simulink model "ps_25V_12kA_r"  (R2026b)
settings: Solver=ode23tb  StopTime=param.sim.simlength  FixedStep=param.glb_time.tc  MaxStep=param.glb_time.tc
values from neighbouring files (symbols this model uses):
  param = struct()    [init_model.m]
undefined symbols (not defined in the file or in its folder): magnitude
libraries: fl_lib x106, nesl_utility x71, afe_uvw_ctrl x5, ee_legacy_lib x5, discrete_time_low_pass_filter x2, three_windings_transformer x2, pi_ctrl x2, threephase_inductor_lib x1, dclink_for_two_levels x1, three_phase_pwm_modulator x1, three_phase_inverter_ideal_switch_based_model x1, three_phase_inverter_igbt_advanced_thermal_model x1
(part 2 of 5)

== system ps_25V_12kA_r/grid/grid_emulator ==
  3ph_Dyg_ssc : Subsystem
  Bus Selector : BusSelector  OutputSignals=ua_grid_emu,ub_grid_emu,uc_grid_emu
  Bus Selector1 : BusSelector  OutputSignals=gamma_grid_emulator,omega_grid_emulator
  Controlled Voltage Source : fl_lib/Electrical/Electrical Sources/Controlled Voltage Source
  Controlled Voltage Source1 : fl_lib/Electrical/Electrical Sources/Controlled Voltage Source
  Controlled Voltage Source2 : fl_lib/Electrical/Electrical Sources/Controlled Voltage Source
  Electrical Reference : fl_lib/Electrical/Electrical Elements/Electrical Reference
  Simulink-PS Converter : nesl_utility/Simulink-PS Converter  PhysicalDomain=network_engine_domain  SubClassName=ps_input  LeftPortType=input  RightPortType=output  PseudoPeriodic=off  Frequencies=[]  NoiseDistribution=none  NoiseParameters=[]  Unit=V  AffineConversion=on  FilteringAndDerivatives=provide  SimscapeFilterOrder=1  InputFilterTimeConstant=0.001  UdotUserProvided=0
  Simulink-PS Converter1 : nesl_utility/Simulink-PS Converter  PhysicalDomain=network_engine_domain  SubClassName=ps_input  LeftPortType=input  RightPortType=output  PseudoPeriodic=off  Frequencies=[]  NoiseDistribution=none  NoiseParameters=[]  Unit=V  AffineConversion=on  FilteringAndDerivatives=provide  SimscapeFilterOrder=1  InputFilterTimeConstant=0.001  UdotUserProvided=0
  Simulink-PS Converter2 : nesl_utility/Simulink-PS Converter  PhysicalDomain=network_engine_domain  SubClassName=ps_input  LeftPortType=input  RightPortType=output  PseudoPeriodic=off  Frequencies=[]  NoiseDistribution=none  NoiseParameters=[]  Unit=V  AffineConversion=on  FilteringAndDerivatives=provide  SimscapeFilterOrder=1  InputFilterTimeConstant=0.001  UdotUserProvided=0
  Solver Configuration : nesl_utility/Solver Configuration  PhysicalDomain=network_engine_domain  SubClassName=solver  LeftPortType=input  RightPortType=generic  Tones=[]  Harmonics=[]  SimulateNoise=off  Profile=off  UseLocalSampling=off  EnableSwitchedLinearOptims=on  FrequencyDomain=off  UseCCode=off  RelTol=0.001  AbsTol=0.001  MinStep=1e-09  ToWorkspace=off  RevertToSquareIcSolve=off  NumHomotopyIterations=100  PhasorMode=off  PhasorModeNumHarmonics=1  ConsistencySolver=NEWTON_FTOL  CanonicalOrdering=UNORDERED  OptimizeIntermediates=UNOPTIMIZED  MulticoreSolverChoice=BACKWARD_EULER  IndexReductionMethod=DerivativeReplacement  DoDC=on  ResidualTolerance=1e-4  ConsistencyTolSource=GLOBAL  ConsistencyAbsTol=0.001  ConsistencyRelTol=0.001  ConsistencyTolFactor=0.001  UseLocalSolver=on  LocalSolverChoice=NE_BACKWARD_EULER_ADVANCER  ResolveIndetEquations=on  FunctionEvalNumThread=1  LocalSolverSampleTime=param.glb_time.tc  DoFixedCost=on  MaxNonlinIter=param.sim.nonlinear_iterations  MaxModeIter=2  ComputeImpulses=off  ImpulseIterations=2  LinearAlgebra=auto  LinearAlgebraNumThread=0  EquationFormulation=NE_TIME_EF  DelaysMemoryBudget=1024  AutomaticFiltering=on  FilteringTimeConstant=0.001  PartitionStorageMethod=AS_NEEDED  PartitionMemoryBudget=1024  PartitionMethod=BALANCED  MultibodyUseLocalSolver=off  MultibodyLocalSolverChoice=ODE1  MultibodyLocalSolverSampleTime=0.001
  td2tc_1 : TransferFcn  Denominator=[param.glb_time.tc 1]
  td2tc_2 : TransferFcn  Denominator=[param.glb_time.tc 1]
  td2tc_3 : TransferFcn  Denominator=[param.glb_time.tc 1]
  three_phase_voltage_source_with_frt_emulator1 : three_phase_voltage_with_frt_emulator_mfcn/three_phase_voltage_source_with_frt_emulator  nominal_frequency_m=param.grid.emu.fgrid_nom  nominal_voltage_m=param.grid.emu.us_secondary_nom  Vemu_ref_norm_m=param.grid.emu.Vemu_ref_norm  vp_xi_pu_m=param.grid.emu.up_xi_pu_ref  vp_eta_pu_m=param.grid.emu.up_eta_pu_ref  vn_xi_pu_m=param.grid.emu.un_xi_pu_ref  vn_eta_pu_m=param.grid.emu.un_eta_pu_ref  Am=param.ctrl.filters.afe.SOF_50Hz.ss_c.A  Bm=param.ctrl.filters.afe.SOF_50Hz.ss_c.B  Cm=param.ctrl.filters.afe.SOF_50Hz.ss_c.C  enable_frt_1_m=param.frt.data.enable_frt_1  enable_frt_2_m=param.frt.data.enable_frt_2  start_time_LVRT_m=param.frt.data.start_time_LVRT  end_time_LVRT_m=param.frt.data.end_time_LVRT  deepPOSxi_m=param.frt.data.deepPOSxi  deepPOSeta_m=param.frt.data.deepPOSeta  deepNEGxi_m=param.frt.data.deepNEGxi  deepNEGeta_m=param.frt.data.deepNEGeta  Amplitude_U_m=param.frt.data.Amplitude_U  Amplitude_V_m=param.frt.data.Amplitude_V  Amplitude_W_m=param.frt.data.Amplitude_W  t_ramp_m=param.frt.data.t_ramp  Phase_shift_m=param.frt.data.Phase_shift
  threephase_vi_measures : Subsystem
  u1 : PMIOPort  Side=Right
  u2 : PMIOPort  Port=2  Side=Right
  u3 : PMIOPort  Port=3  Side=Right
  tag scope: omega_grid_emulator=global, phase_grid_emulator=global
  wires:
  Bus Selector1/2 -> [omega_grid_emulator]  "<omega_grid_emulator>"
  Bus Selector1/1 -> [phase_grid_emulator]  "<gamma_grid_emulator>"
  Bus Selector/2 -> td2tc_2/1  "<ub_grid_emu>"
  Bus Selector/3 -> td2tc_3/1  "<uc_grid_emu>"
  three_phase_voltage_source_with_frt_emulator1/1 -> Bus Selector1/1, Bus Selector/1
  Bus Selector/1 -> td2tc_1/1  "<ua_grid_emu>"
  td2tc_1/1 -> Simulink-PS Converter/1  "ua(t)"
  td2tc_2/1 -> Simulink-PS Converter1/1  "ub(t)"
  td2tc_3/1 -> Simulink-PS Converter2/1  "uc(t)"
  connections:
  Simulink-PS Converter/RConn1 -- Controlled Voltage Source/RConn1
  Simulink-PS Converter1/RConn1 -- Controlled Voltage Source1/RConn1
  Simulink-PS Converter2/RConn1 -- Controlled Voltage Source2/RConn1
  Controlled Voltage Source/RConn2 -- Controlled Voltage Source1/RConn2 -- Controlled Voltage Source2/RConn2 -- Electrical Reference/LConn1 -- Solver Configuration/RConn1
  3ph_Dyg_ssc/RConn1 -- u1/RConn1
  3ph_Dyg_ssc/RConn2 -- u2/RConn1
  3ph_Dyg_ssc/RConn3 -- u3/RConn1
  3ph_Dyg_ssc/LConn1 -- threephase_vi_measures/RConn1
  3ph_Dyg_ssc/LConn2 -- threephase_vi_measures/RConn2
  3ph_Dyg_ssc/LConn3 -- threephase_vi_measures/RConn3
  Controlled Voltage Source/LConn1 -- threephase_vi_measures/LConn1
  Controlled Voltage Source1/LConn1 -- threephase_vi_measures/LConn2
  Controlled Voltage Source2/LConn1 -- threephase_vi_measures/LConn3

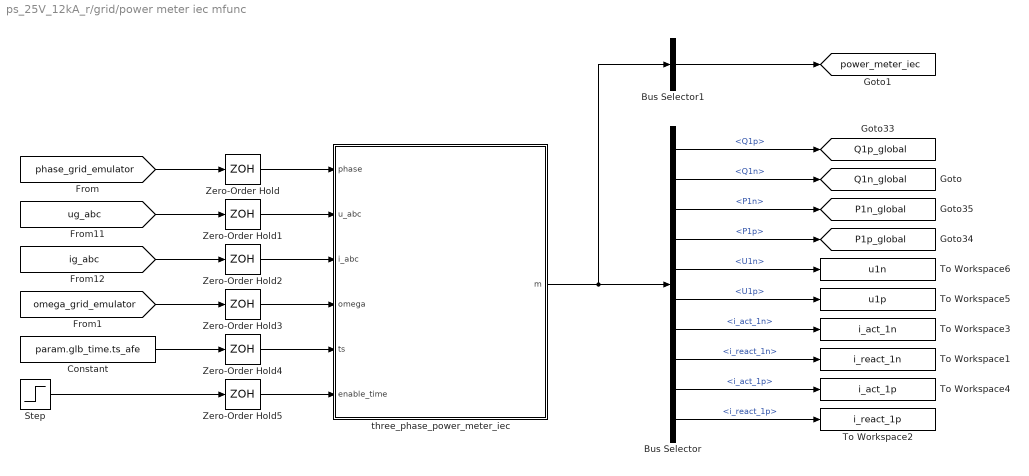
== system ps_25V_12kA_r/grid/power meter iec mfunc ==
  Bus Selector : BusSelector  OutputSignals=Q1p,Q1n,P1n,P1p,U1n,U1p,i_act_1n,i_react_1n,i_act_1p,i_react_1p
  Bus Selector1 : BusSelector  OutputSignals=Q1p,Q1n,P1n,P1p  OutputAsBus=on
  Constant : Constant  Value=param.glb_time.ts_afe
  Step : Step  Time=0.025  InitialValue=1  FinalValue=0  SampleTime=0
  To Workspace1 : ToWorkspace  VariableName=i_react_1n  SampleTime=param.glb_time.ts_afe
      settings: MaxDataPoints=param.glb_time.Ns_afe
  To Workspace2 : ToWorkspace  VariableName=i_react_1p  SampleTime=param.glb_time.ts_afe
      settings: MaxDataPoints=param.glb_time.Ns_afe
  To Workspace3 : ToWorkspace  VariableName=i_act_1n  SampleTime=param.glb_time.ts_afe
      settings: MaxDataPoints=param.glb_time.Ns_afe
  To Workspace4 : ToWorkspace  VariableName=i_act_1p  SampleTime=param.glb_time.ts_afe
      settings: MaxDataPoints=param.glb_time.Ns_afe
  To Workspace5 : ToWorkspace  VariableName=u1p  SampleTime=param.glb_time.ts_afe
      settings: MaxDataPoints=param.glb_time.Ns_afe
  To Workspace6 : ToWorkspace  VariableName=u1n  SampleTime=param.glb_time.ts_afe
      settings: MaxDataPoints=param.glb_time.Ns_afe
  Zero-Order Hold{,1..5} (6 alike) : ZeroOrderHold  SampleTime=param.glb_time.ts_afe
  three_phase_power_meter_iec : MATLAB Function  TreatAsAtomicUnit=on  SystemSampleTime=param.glb_time.ts_afe
  tag scope: P1n_global=global, P1p_global=global, Q1n_global=global, Q1p_global=global, power_meter_iec=global
  wires:
  Bus Selector/6 -> To Workspace5/1  "<U1p>"
  Bus Selector/8 -> To Workspace1/1  "<i_react_1n>"
  Bus Selector/10 -> To Workspace2/1  "<i_react_1p>"
  Bus Selector/5 -> To Workspace6/1  "<U1n>"
  Bus Selector/4 -> [P1p_global]  "<P1p>"
  Bus Selector/2 -> [Q1n_global]  "<Q1n>"
  Bus Selector/1 -> [Q1p_global]  "<Q1p>"
  Bus Selector/7 -> To Workspace3/1  "<i_act_1n>"
  Bus Selector/9 -> To Workspace4/1  "<i_act_1p>"
  Bus Selector/3 -> [P1n_global]  "<P1n>"
  three_phase_power_meter_iec/1(m) -> Bus Selector1/1, Bus Selector/1
  Zero-Order Hold/1 -> three_phase_power_meter_iec/1(phase)
  Zero-Order Hold2/1 -> three_phase_power_meter_iec/3(i_abc)
  [phase_grid_emulator] -> Zero-Order Hold/1
  Step/1 -> Zero-Order Hold5/1
  Zero-Order Hold3/1 -> three_phase_power_meter_iec/4(omega)
  Zero-Order Hold4/1 -> three_phase_power_meter_iec/5(ts)
  [ug_abc] -> Zero-Order Hold1/1
  Zero-Order Hold5/1 -> three_phase_power_meter_iec/6(enable_time)
  [ig_abc] -> Zero-Order Hold2/1
  [omega_grid_emulator] -> Zero-Order Hold3/1
  Constant/1 -> Zero-Order Hold4/1
  Zero-Order Hold1/1 -> three_phase_power_meter_iec/2(u_abc)
  Bus Selector1/1 -> [power_meter_iec]

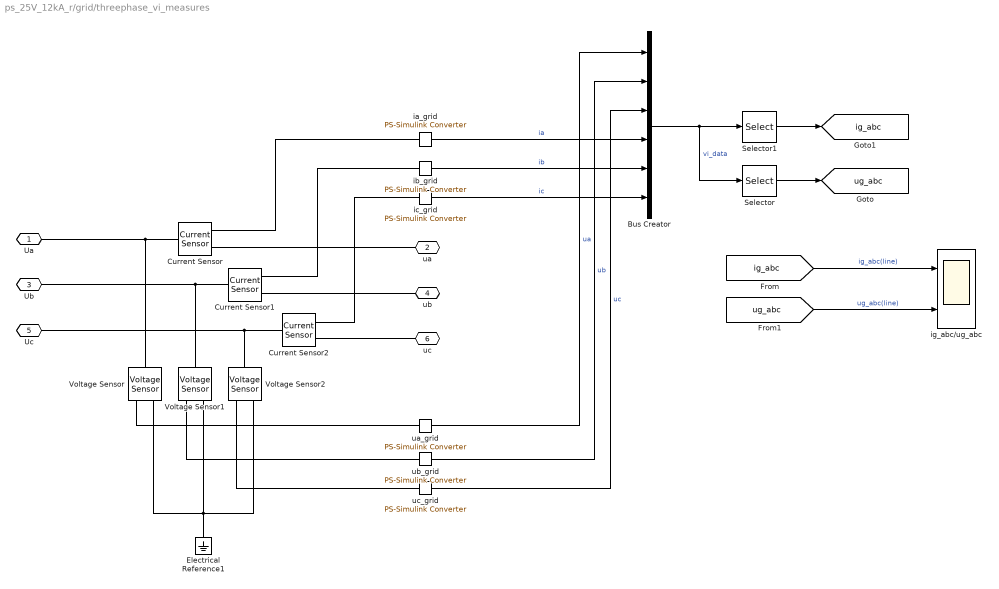
== system ps_25V_12kA_r/grid/threephase_vi_measures ==
  Bus Creator : BusCreator  Inputs=6
  Current Sensor : fl_lib/Electrical/Electrical Sensors/Current Sensor
  Current Sensor1 : fl_lib/Electrical/Electrical Sensors/Current Sensor
  Current Sensor2 : fl_lib/Electrical/Electrical Sensors/Current Sensor
  Electrical Reference1 : fl_lib/Electrical/Electrical Elements/Electrical Reference
  Selector : Selector  InputPortWidth=6  IndexOptions=Index vector (dialog)  Indices=[1 2 3]  OutputSizes=1  RuntimeRangeChecks=off
  Selector1 : Selector  InputPortWidth=6  IndexOptions=Index vector (dialog)  Indices=[4 5 6]  OutputSizes=1  RuntimeRangeChecks=off
  Voltage Sensor : fl_lib/Electrical/Electrical Sensors/Voltage Sensor
  Voltage Sensor1 : fl_lib/Electrical/Electrical Sensors/Voltage Sensor
  Voltage Sensor2 : fl_lib/Electrical/Electrical Sensors/Voltage Sensor
  ia_grid : nesl_utility/PS-Simulink Converter  PhysicalDomain=network_engine_domain  SubClassName=ps_output  LeftPortType=input  RightPortType=output  PseudoPeriodic=off  Frequencies=[]  VectorFormat=1-D array  Unit=A  AffineConversion=off
  ib_grid : nesl_utility/PS-Simulink Converter  PhysicalDomain=network_engine_domain  SubClassName=ps_output  LeftPortType=input  RightPortType=output  PseudoPeriodic=off  Frequencies=[]  VectorFormat=1-D array  Unit=A  AffineConversion=off
  ic_grid : nesl_utility/PS-Simulink Converter  PhysicalDomain=network_engine_domain  SubClassName=ps_output  LeftPortType=input  RightPortType=output  PseudoPeriodic=off  Frequencies=[]  VectorFormat=1-D array  Unit=A  AffineConversion=off
  ig_abc/ug_abc : Scope  NumInputPorts=2
      settings: SampleTime=param.glb_time.tc  ActiveDisplayYMinimum=-728.92703752654245  ActiveDisplayYMaximum=734.90808013997  DataLoggingVariableName=ScopeData2
  ua_grid : nesl_utility/PS-Simulink Converter  PhysicalDomain=network_engine_domain  SubClassName=ps_output  LeftPortType=input  RightPortType=output  PseudoPeriodic=off  Frequencies=[]  VectorFormat=1-D array  Unit=V  AffineConversion=off
  ub_grid : nesl_utility/PS-Simulink Converter  PhysicalDomain=network_engine_domain  SubClassName=ps_output  LeftPortType=input  RightPortType=output  PseudoPeriodic=off  Frequencies=[]  VectorFormat=1-D array  Unit=V  AffineConversion=off
  uc_grid : nesl_utility/PS-Simulink Converter  PhysicalDomain=network_engine_domain  SubClassName=ps_output  LeftPortType=input  RightPortType=output  PseudoPeriodic=off  Frequencies=[]  VectorFormat=1-D array  Unit=V  AffineConversion=off
  Ua : PMIOPort  Side=Left
  ua : PMIOPort  Port=2  Side=Right
  Ub : PMIOPort  Port=3  Side=Left
  ub : PMIOPort  Port=4  Side=Right
  Uc : PMIOPort  Port=5  Side=Left
  uc : PMIOPort  Port=6  Side=Right
  tag scope: ig_abc=global, ug_abc=global
  wires:
  Bus Creator/1 -> Selector1/1, Selector/1  "vi_data"
  Selector/1 -> [ug_abc]
  ib_grid/1 -> Bus Creator/5  "ib"
  ia_grid/1 -> Bus Creator/4  "ia"
  ic_grid/1 -> Bus Creator/6  "ic"
  ua_grid/1 -> Bus Creator/1  "ua"
  ub_grid/1 -> Bus Creator/2  "ub"
  uc_grid/1 -> Bus Creator/3  "uc"
  Selector1/1 -> [ig_abc]
  [ug_abc] -> ig_abc/ug_abc/2  "ug_abc(line)"
  [ig_abc] -> ig_abc/ug_abc/1  "ig_abc(line)"
  connections:
  Current Sensor1/LConn1 -- Ub/RConn1 -- Voltage Sensor1/LConn1
  Electrical Reference1/LConn1 -- Voltage Sensor/RConn2 -- Voltage Sensor2/RConn2 -- Voltage Sensor1/RConn2
  Voltage Sensor/RConn1 -- ua_grid/LConn1
  Current Sensor/RConn2 -- ua/RConn1
  Voltage Sensor1/RConn1 -- ub_grid/LConn1
  Voltage Sensor2/LConn1 -- Current Sensor2/LConn1 -- Uc/RConn1
  Current Sensor/LConn1 -- Ua/RConn1 -- Voltage Sensor/LConn1
  Current Sensor1/RConn2 -- ub/RConn1
  Voltage Sensor2/RConn1 -- uc_grid/LConn1
  ib_grid/LConn1 -- Current Sensor1/RConn1
  ia_grid/LConn1 -- Current Sensor/RConn1
  ic_grid/LConn1 -- Current Sensor2/RConn1
  Current Sensor2/RConn2 -- uc/RConn1

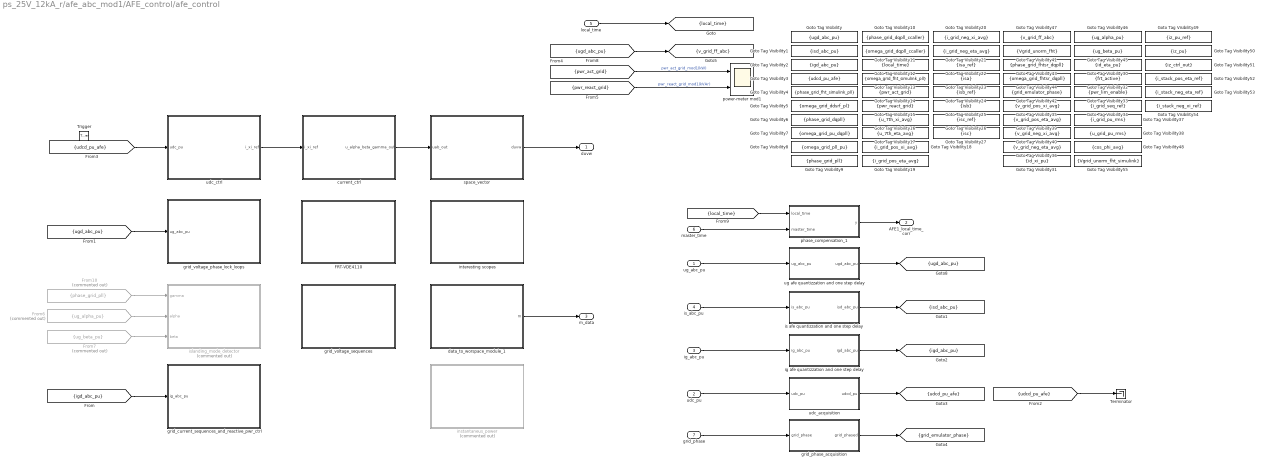
== system ps_25V_12kA_r/afe_abc_mod1/AFE_control/afe_control ==
  ug_abc_pu : Inport
  udc_pu : Inport  Port=2
  ig_abc_pu : Inport  Port=3
  is_abc_pu : Inport  Port=4
  local_time : Inport  Port=5
  master_time : Inport  Port=6
  grid_phase : Inport  Port=7
  Trigger : TriggerPort  VariantControl=(inherit)  PortDimensions=1
  FRT-VDE4110 : Subsystem
  From10 : From  Commented=on  GotoTag=phase_grid_pll
  From6 : From  Commented=on  GotoTag=ug_alpha_pu
  From7 : From  Commented=on  GotoTag=ug_beta_pu
  Goto Tag Visibility : GotoTagVisibility  GotoTag=ugd_abc_pu
  Goto Tag Visibility1 : GotoTagVisibility  GotoTag=isd_abc_pu
  Goto Tag Visibility10 : GotoTagVisibility  GotoTag=phase_grid_dqpll_ccaller
  Goto Tag Visibility11 : GotoTagVisibility  GotoTag=omega_grid_dqpll_ccaller
  Goto Tag Visibility12 : GotoTagVisibility  GotoTag=local_time
  Goto Tag Visibility13 : GotoTagVisibility  GotoTag=omega_grid_fht_simulink_pll
  Goto Tag Visibility14 : GotoTagVisibility  GotoTag=pwr_act_grid
  Goto Tag Visibility15 : GotoTagVisibility  GotoTag=pwr_react_grid
  Goto Tag Visibility16 : GotoTagVisibility  GotoTag=u_7th_xi_avg
  Goto Tag Visibility17 : GotoTagVisibility  GotoTag=u_7th_eta_avg
  Goto Tag Visibility18 : GotoTagVisibility  GotoTag=i_grid_pos_xi_avg
  Goto Tag Visibility19 : GotoTagVisibility  GotoTag=i_grid_pos_eta_avg
  Goto Tag Visibility2 : GotoTagVisibility  GotoTag=igd_abc_pu
  Goto Tag Visibility20 : GotoTagVisibility  GotoTag=i_grid_neg_xi_avg
  Goto Tag Visibility21 : GotoTagVisibility  GotoTag=i_grid_neg_eta_avg
  Goto Tag Visibility22 : GotoTagVisibility  GotoTag=isa_ref
  Goto Tag Visibility23 : GotoTagVisibility  GotoTag=isa
  Goto Tag Visibility24 : GotoTagVisibility  GotoTag=isb_ref
  Goto Tag Visibility25 : GotoTagVisibility  GotoTag=isb
  Goto Tag Visibility26 : GotoTagVisibility  GotoTag=isc_ref
  Goto Tag Visibility27 : GotoTagVisibility  GotoTag=isc
  Goto Tag Visibility3 : GotoTagVisibility  GotoTag=udcd_pu_afe
  Goto Tag Visibility30 : GotoTagVisibility  GotoTag=id_eta_pu
  Goto Tag Visibility31 : GotoTagVisibility  GotoTag=id_xi_pu
  Goto Tag Visibility32 : GotoTagVisibility  GotoTag=frt_active
  Goto Tag Visibility33 : GotoTagVisibility  GotoTag=pwr_lim_enable
  Goto Tag Visibility34 : GotoTagVisibility  GotoTag=i_grid_seq_ref
  Goto Tag Visibility35 : GotoTagVisibility  GotoTag=v_grid_pos_xi_avg
  Goto Tag Visibility36 : GotoTagVisibility  GotoTag=v_grid_neg_eta_avg
  Goto Tag Visibility37 : GotoTagVisibility  GotoTag=i_grid_pu_rms
  Goto Tag Visibility38 : GotoTagVisibility  GotoTag=u_grid_pu_rms
  Goto Tag Visibility39 : GotoTagVisibility  GotoTag=v_grid_pos_eta_avg
  Goto Tag Visibility4 : GotoTagVisibility  GotoTag=phase_grid_fht_simulink_pll
  Goto Tag Visibility40 : GotoTagVisibility  GotoTag=v_grid_neg_xi_avg
  Goto Tag Visibility41 : GotoTagVisibility  GotoTag=Vgrid_unorm_fht
  Goto Tag Visibility42 : GotoTagVisibility  GotoTag=grid_emulator_phase
  Goto Tag Visibility43 : GotoTagVisibility  GotoTag=phase_grid_fhtsr_dqpll
  Goto Tag Visibility44 : GotoTagVisibility  GotoTag=omega_grid_fhtsr_dqpll
  Goto Tag Visibility45 : GotoTagVisibility  GotoTag=ug_beta_pu
  Goto Tag Visibility46 : GotoTagVisibility  GotoTag=ug_alpha_pu
  Goto Tag Visibility47 : GotoTagVisibility  GotoTag=v_grid_ff_abc
  Goto Tag Visibility48 : GotoTagVisibility  GotoTag=cos_phi_avg
  Goto Tag Visibility49 : GotoTagVisibility  GotoTag=iz_pu_ref
  Goto Tag Visibility5 : GotoTagVisibility  GotoTag=omega_grid_ddsrf_pl
  Goto Tag Visibility50 : GotoTagVisibility  GotoTag=iz_pu
  Goto Tag Visibility51 : GotoTagVisibility  GotoTag=iz_ctrl_out
  Goto Tag Visibility52 : GotoTagVisibility  GotoTag=i_stack_pos_eta_ref
  Goto Tag Visibility53 : GotoTagVisibility  GotoTag=i_stack_neg_eta_ref
  Goto Tag Visibility54 : GotoTagVisibility  GotoTag=i_stack_neg_xi_ref
  Goto Tag Visibility55 : GotoTagVisibility  GotoTag=Vgrid_unorm_fht_simulink
  Goto Tag Visibility6 : GotoTagVisibility  GotoTag=phase_grid_dqpll
  Goto Tag Visibility7 : GotoTagVisibility  GotoTag=omega_grid_pu_dqpll
  Goto Tag Visibility8 : GotoTagVisibility  GotoTag=omega_grid_pll_pu
  Goto Tag Visibility9 : GotoTagVisibility  GotoTag=phase_grid_pll
  Terminator : Terminator
  current_ctrl : Subsystem
  data_to_worspace_module_1 : Subsystem
  grid_current_sequences_and_reactive_pwr_ctrl : Subsystem
  grid_phase_acquisition : Subsystem
  grid_voltage_phase_lock_loops : Subsystem
  grid_voltage_sequences : Subsystem
  ig afe quantizzation and one step delay : Subsystem
  instantaneus_power : Subsystem  Commented=on
  interesting scopes : Subsystem
  is afe quantizzation and one step delay : Subsystem
  islanding_mode_detector : Subsystem  Commented=on
  phase_compensation_1 : Subsystem
  power-meter mod1 : Scope  NumInputPorts=2
      settings: ActiveDisplayYMinimum=-67.030069207436668  ActiveDisplayYMaximum=116.57466656594397  DataLoggingVariableName=ScopeData9
  space_vector : Subsystem
  udc_acquisition : Subsystem
  udc_ctrl : Subsystem
  ug afe quantizzation and one step delay : Subsystem
  duvw : Outport
  AFE1_local_time_corr : Outport  Port=2
  m_data : Outport  Port=3
  tag scope: grid_emulator_phase=scoped, igd_abc_pu=scoped, isd_abc_pu=scoped, local_time=scoped, udcd_pu_afe=scoped, ugd_abc_pu=scoped, v_grid_ff_abc=scoped
  wires:
  ug_abc_pu/1 -> ug afe quantizzation and one step delay/1(ug_abc_pu)
  space_vector/1(duvw) -> duvw/1
  is_abc_pu/1 -> is afe quantizzation and one step delay/1(is_abc_pu)
  ig_abc_pu/1 -> ig afe quantizzation and one step delay/1(ig_abc_pu)
  [ugd_abc_pu] -> grid_voltage_phase_lock_loops/1(ug_abc_pu)
  [igd_abc_pu] -> grid_current_sequences_and_reactive_pwr_ctrl/1(ig_abc_pu)
  [udcd_pu_afe] -> udc_ctrl/1(udc_pu)
  udc_pu/1 -> udc_acquisition/1(udc_pu)
  udc_acquisition/1(udcd_pu) -> [udcd_pu_afe]
  [pwr_react_grid] -> power-meter mod1/2  "pwr_react_grid_mod1(kVAr)"
  [pwr_act_grid] -> power-meter mod1/1  "pwr_act_grid_mod1(kW)"
  From10/1 -> islanding_mode_detector/1(gamma)
  From6/1 -> islanding_mode_detector/2(alpha)
  ug afe quantizzation and one step delay/1(ugd_abc_pu) -> [ugd_abc_pu]
  is afe quantizzation and one step delay/1(isd_abc_pu) -> [isd_abc_pu]
  ig afe quantizzation and one step delay/1(igd_abc_pu) -> [igd_abc_pu]
  From7/1 -> islanding_mode_detector/3(beta)
  local_time/1 -> [local_time]
  master_time/1 -> phase_compensation_1/2(master_time)
  phase_compensation_1/1(y) -> AFE1_local_time_corr/1
  [local_time] -> phase_compensation_1/1(local_time)
  grid_phase/1 -> grid_phase_acquisition/1(grid_phase)
  grid_phase_acquisition/1(grid_phased) -> [grid_emulator_phase]
  [ugd_abc_pu] -> [v_grid_ff_abc]
  data_to_worspace_module_1/1(m) -> m_data/1
  [udcd_pu_afe] -> Terminator/1
  udc_ctrl/1(i_xi_ref) -> current_ctrl/1(i_xi_ref)
  current_ctrl/1(u_alpha_beta_gamma_out) -> space_vector/1(uab_out)

== system ps_25V_12kA_r/afe_abc_mod1/LCL_filter/CapacitorFilter ==
  CFu1 : fl_lib/Electrical/Electrical Elements/Capacitor  c=param.afe.hw.CFu F  r=param.afe.hw.RCFu Ohm  g=0 1/Ohm  i_specify=off  i_priority=None  i=0 A  i_nominal_specify=off  i_nominal_value=1  i_nominal_unit=A  v_specify=off  v_priority=None  v=0 V  v_nominal_specify=off  v_nominal_value=1  v_nominal_unit=V  vc_specify=off  vc_priority=High  vc=0 V  vc_nominal_specify=off  vc_nominal_value=1  vc_nominal_unit=V
  CFu2 : fl_lib/Electrical/Electrical Elements/Capacitor  c=param.afe.hw.CFu F  r=param.afe.hw.RCFu Ohm  g=0 1/Ohm  i_specify=off  i_priority=None  i=0 A  i_nominal_specify=off  i_nominal_value=1  i_nominal_unit=A  v_specify=off  v_priority=None  v=0 V  v_nominal_specify=off  v_nominal_value=1  v_nominal_unit=V  vc_specify=off  vc_priority=High  vc=0 V  vc_nominal_specify=off  vc_nominal_value=1  vc_nominal_unit=V
  CFu3 : fl_lib/Electrical/Electrical Elements/Capacitor  c=param.afe.hw.CFu F  r=param.afe.hw.RCFu Ohm  g=0 1/Ohm  i_specify=off  i_priority=None  i=0 A  i_nominal_specify=off  i_nominal_value=1  i_nominal_unit=A  v_specify=off  v_priority=None  v=0 V  v_nominal_specify=off  v_nominal_value=1  v_nominal_unit=V  vc_specify=off  vc_priority=High  vc=0 V  vc_nominal_specify=off  vc_nominal_value=1  vc_nominal_unit=V
  Current Sensor : fl_lib/Electrical/Electrical Sensors/Current Sensor
  Current Sensor1 : fl_lib/Electrical/Electrical Sensors/Current Sensor
  Current Sensor2 : fl_lib/Electrical/Electrical Sensors/Current Sensor
  iu_CFu : nesl_utility/PS-Simulink Converter  PhysicalDomain=network_engine_domain  SubClassName=ps_output  LeftPortType=input  RightPortType=output  PseudoPeriodic=off  Frequencies=[]  VectorFormat=1-D array  Unit=A  AffineConversion=off
  iv_CFu : nesl_utility/PS-Simulink Converter  PhysicalDomain=network_engine_domain  SubClassName=ps_output  LeftPortType=input  RightPortType=output  PseudoPeriodic=off  Frequencies=[]  VectorFormat=1-D array  Unit=A  AffineConversion=off
  iw_CFu : nesl_utility/PS-Simulink Converter  PhysicalDomain=network_engine_domain  SubClassName=ps_output  LeftPortType=input  RightPortType=output  PseudoPeriodic=off  Frequencies=[]  VectorFormat=1-D array  Unit=A  AffineConversion=off
  u : PMIOPort  Side=Left
  v : PMIOPort  Port=2  Side=Left
  w : PMIOPort  Port=3  Side=Left
  tag scope: icu_CFu_mod1=global, icv_CFu_mod1=global, icw_CFu_mod1=global
  wires:
  iw_CFu/1 -> [icw_CFu_mod1]
  iv_CFu/1 -> [icv_CFu_mod1]
  iu_CFu/1 -> [icu_CFu_mod1]
  connections:
  Current Sensor/RConn2 -- CFu3/LConn1
  Current Sensor/RConn1 -- iw_CFu/LConn1
  CFu1/RConn1 -- CFu3/RConn1 -- CFu2/RConn1
  Current Sensor/LConn1 -- w/RConn1
  Current Sensor1/RConn2 -- CFu2/LConn1
  Current Sensor1/RConn1 -- iv_CFu/LConn1
  Current Sensor1/LConn1 -- v/RConn1
  Current Sensor2/LConn1 -- u/RConn1
  Current Sensor2/RConn1 -- iu_CFu/LConn1
  CFu1/LConn1 -- Current Sensor2/RConn2

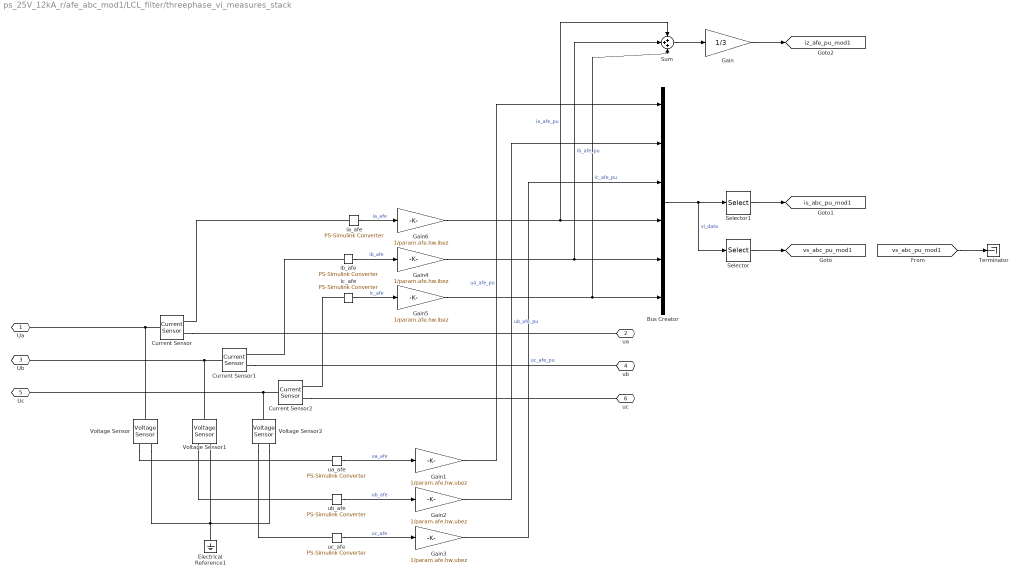
== system ps_25V_12kA_r/afe_abc_mod1/LCL_filter/threephase_vi_measures_stack ==
  Bus Creator : BusCreator  Inputs=6
  Current Sensor : fl_lib/Electrical/Electrical Sensors/Current Sensor
  Current Sensor1 : fl_lib/Electrical/Electrical Sensors/Current Sensor
  Current Sensor2 : fl_lib/Electrical/Electrical Sensors/Current Sensor
  Electrical Reference1 : fl_lib/Electrical/Electrical Elements/Electrical Reference
  Gain : Gain  Gain=1/3
  Gain1 : Gain  Gain=1/param.afe.hw.ubez
  Gain2 : Gain  Gain=1/param.afe.hw.ubez
  Gain3 : Gain  Gain=1/param.afe.hw.ubez
  Gain4 : Gain  Gain=1/param.afe.hw.ibez
  Gain5 : Gain  Gain=1/param.afe.hw.ibez
  Gain6 : Gain  Gain=1/param.afe.hw.ibez
  Selector : Selector  InputPortWidth=6  IndexOptions=Index vector (dialog)  Indices=[1 2 3]  OutputSizes=1  RuntimeRangeChecks=off
  Selector1 : Selector  InputPortWidth=6  IndexOptions=Index vector (dialog)  Indices=[4 5 6]  OutputSizes=1  RuntimeRangeChecks=off
  Sum : Sum  Inputs=+++
  Terminator : Terminator
  Voltage Sensor : fl_lib/Electrical/Electrical Sensors/Voltage Sensor
  Voltage Sensor1 : fl_lib/Electrical/Electrical Sensors/Voltage Sensor
  Voltage Sensor2 : fl_lib/Electrical/Electrical Sensors/Voltage Sensor
  ia_afe : nesl_utility/PS-Simulink Converter  PhysicalDomain=network_engine_domain  SubClassName=ps_output  LeftPortType=input  RightPortType=output  PseudoPeriodic=off  Frequencies=[]  VectorFormat=1-D array  Unit=A  AffineConversion=off
  ib_afe : nesl_utility/PS-Simulink Converter  PhysicalDomain=network_engine_domain  SubClassName=ps_output  LeftPortType=input  RightPortType=output  PseudoPeriodic=off  Frequencies=[]  VectorFormat=1-D array  Unit=A  AffineConversion=off
  ic_afe : nesl_utility/PS-Simulink Converter  PhysicalDomain=network_engine_domain  SubClassName=ps_output  LeftPortType=input  RightPortType=output  PseudoPeriodic=off  Frequencies=[]  VectorFormat=1-D array  Unit=A  AffineConversion=off
  ua_afe : nesl_utility/PS-Simulink Converter  PhysicalDomain=network_engine_domain  SubClassName=ps_output  LeftPortType=input  RightPortType=output  PseudoPeriodic=off  Frequencies=[]  VectorFormat=1-D array  Unit=V  AffineConversion=off
  ub_afe : nesl_utility/PS-Simulink Converter  PhysicalDomain=network_engine_domain  SubClassName=ps_output  LeftPortType=input  RightPortType=output  PseudoPeriodic=off  Frequencies=[]  VectorFormat=1-D array  Unit=V  AffineConversion=off
  uc_afe : nesl_utility/PS-Simulink Converter  PhysicalDomain=network_engine_domain  SubClassName=ps_output  LeftPortType=input  RightPortType=output  PseudoPeriodic=off  Frequencies=[]  VectorFormat=1-D array  Unit=V  AffineConversion=off
  Ua : PMIOPort  Side=Left
  ua : PMIOPort  Port=2  Side=Right
  Ub : PMIOPort  Port=3  Side=Left
  ub : PMIOPort  Port=4  Side=Right
  Uc : PMIOPort  Port=5  Side=Left
  uc : PMIOPort  Port=6  Side=Right
  tag scope: is_abc_pu_mod1=global, iz_afe_pu_mod1=global, vs_abc_pu_mod1=global
  wires:
  Bus Creator/1 -> Selector/1, Selector1/1  "vi_data"
  Selector/1 -> [vs_abc_pu_mod1]
  ib_afe/1 -> Gain4/1  "ib_afe"
  ia_afe/1 -> Gain6/1  "ia_afe"
  ic_afe/1 -> Gain5/1  "ic_afe"
  ua_afe/1 -> Gain1/1  "ua_afe"
  ub_afe/1 -> Gain2/1  "ub_afe"
  uc_afe/1 -> Gain3/1  "uc_afe"
  Selector1/1 -> [is_abc_pu_mod1]
  Sum/1 -> Gain/1
  Gain/1 -> [iz_afe_pu_mod1]
  Gain1/1 -> Bus Creator/1  "ua_afe_pu"
  Gain2/1 -> Bus Creator/2  "ub_afe_pu"
  Gain3/1 -> Bus Creator/3  "uc_afe_pu"
  Gain6/1 -> Sum/1, Bus Creator/4  "ia_afe_pu"
  Gain4/1 -> Sum/2, Bus Creator/5  "ib_afe_pu"
  Gain5/1 -> Bus Creator/6, Sum/3  "ic_afe_pu"
  [vs_abc_pu_mod1] -> Terminator/1
  connections:
  Current Sensor1/LConn1 -- Ub/RConn1 -- Voltage Sensor1/LConn1
  Electrical Reference1/LConn1 -- Voltage Sensor/RConn2 -- Voltage Sensor2/RConn2 -- Voltage Sensor1/RConn2
  Voltage Sensor/RConn1 -- ua_afe/LConn1
  Current Sensor/RConn2 -- ua/RConn1
  Voltage Sensor1/RConn1 -- ub_afe/LConn1
  Voltage Sensor2/LConn1 -- Uc/RConn1 -- Current Sensor2/LConn1
  Current Sensor/LConn1 -- Ua/RConn1 -- Voltage Sensor/LConn1
  Current Sensor1/RConn2 -- ub/RConn1
  Voltage Sensor2/RConn1 -- uc_afe/LConn1
  ib_afe/LConn1 -- Current Sensor1/RConn1
  ia_afe/LConn1 -- Current Sensor/RConn1
  ic_afe/LConn1 -- Current Sensor2/RConn1
  Current Sensor2/RConn2 -- uc/RConn1

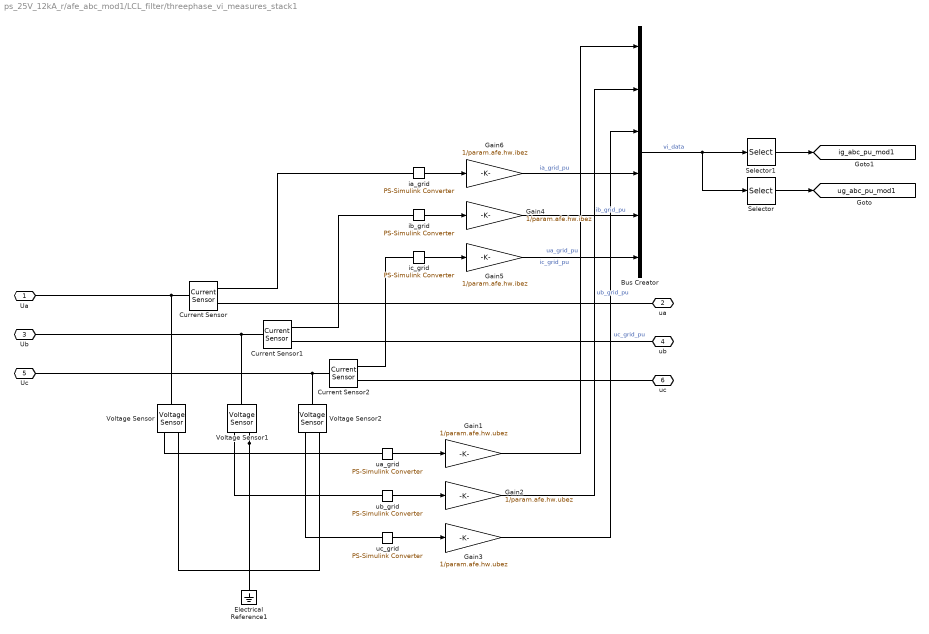
== system ps_25V_12kA_r/afe_abc_mod1/LCL_filter/threephase_vi_measures_stack1 ==
  Bus Creator : BusCreator  Inputs=6
  Current Sensor : fl_lib/Electrical/Electrical Sensors/Current Sensor
  Current Sensor1 : fl_lib/Electrical/Electrical Sensors/Current Sensor
  Current Sensor2 : fl_lib/Electrical/Electrical Sensors/Current Sensor
  Electrical Reference1 : fl_lib/Electrical/Electrical Elements/Electrical Reference
  Gain1 : Gain  Gain=1/param.afe.hw.ubez
  Gain2 : Gain  Gain=1/param.afe.hw.ubez
  Gain3 : Gain  Gain=1/param.afe.hw.ubez
  Gain4 : Gain  Gain=1/param.afe.hw.ibez
  Gain5 : Gain  Gain=1/param.afe.hw.ibez
  Gain6 : Gain  Gain=1/param.afe.hw.ibez
  Selector : Selector  InputPortWidth=6  IndexOptions=Index vector (dialog)  Indices=[1 2 3]  OutputSizes=1  RuntimeRangeChecks=off
  Selector1 : Selector  InputPortWidth=6  IndexOptions=Index vector (dialog)  Indices=[4 5 6]  OutputSizes=1  RuntimeRangeChecks=off
  Voltage Sensor : fl_lib/Electrical/Electrical Sensors/Voltage Sensor
  Voltage Sensor1 : fl_lib/Electrical/Electrical Sensors/Voltage Sensor
  Voltage Sensor2 : fl_lib/Electrical/Electrical Sensors/Voltage Sensor
  ia_grid : nesl_utility/PS-Simulink Converter  PhysicalDomain=network_engine_domain  SubClassName=ps_output  LeftPortType=input  RightPortType=output  PseudoPeriodic=off  Frequencies=[]  VectorFormat=1-D array  Unit=A  AffineConversion=off
  ib_grid : nesl_utility/PS-Simulink Converter  PhysicalDomain=network_engine_domain  SubClassName=ps_output  LeftPortType=input  RightPortType=output  PseudoPeriodic=off  Frequencies=[]  VectorFormat=1-D array  Unit=A  AffineConversion=off
  ic_grid : nesl_utility/PS-Simulink Converter  PhysicalDomain=network_engine_domain  SubClassName=ps_output  LeftPortType=input  RightPortType=output  PseudoPeriodic=off  Frequencies=[]  VectorFormat=1-D array  Unit=A  AffineConversion=off
  ua_grid : nesl_utility/PS-Simulink Converter  PhysicalDomain=network_engine_domain  SubClassName=ps_output  LeftPortType=input  RightPortType=output  PseudoPeriodic=off  Frequencies=[]  VectorFormat=1-D array  Unit=V  AffineConversion=off
  ub_grid : nesl_utility/PS-Simulink Converter  PhysicalDomain=network_engine_domain  SubClassName=ps_output  LeftPortType=input  RightPortType=output  PseudoPeriodic=off  Frequencies=[]  VectorFormat=1-D array  Unit=V  AffineConversion=off
  uc_grid : nesl_utility/PS-Simulink Converter  PhysicalDomain=network_engine_domain  SubClassName=ps_output  LeftPortType=input  RightPortType=output  PseudoPeriodic=off  Frequencies=[]  VectorFormat=1-D array  Unit=V  AffineConversion=off
  Ua : PMIOPort  Side=Left
  ua : PMIOPort  Port=2  Side=Right
  Ub : PMIOPort  Port=3  Side=Left
  ub : PMIOPort  Port=4  Side=Right
  Uc : PMIOPort  Port=5  Side=Left
  uc : PMIOPort  Port=6  Side=Right
  tag scope: ig_abc_pu_mod1=global, ug_abc_pu_mod1=global
  wires:
  Selector1/1 -> [ig_abc_pu_mod1]
  uc_grid/1 -> Gain3/1
  ub_grid/1 -> Gain2/1
  ua_grid/1 -> Gain1/1
  ic_grid/1 -> Gain5/1
  ia_grid/1 -> Gain6/1
  ib_grid/1 -> Gain4/1
  Selector/1 -> [ug_abc_pu_mod1]
  Bus Creator/1 -> Selector1/1, Selector/1  "vi_data"
  Gain1/1 -> Bus Creator/1  "ua_grid_pu"
  Gain2/1 -> Bus Creator/2  "ub_grid_pu"
  Gain3/1 -> Bus Creator/3  "uc_grid_pu"
  Gain6/1 -> Bus Creator/4  "ia_grid_pu"
  Gain4/1 -> Bus Creator/5  "ib_grid_pu"
  Gain5/1 -> Bus Creator/6  "ic_grid_pu"
  connections:
  Current Sensor2/RConn2 -- uc/RConn1
  ic_grid/LConn1 -- Current Sensor2/RConn1
  ia_grid/LConn1 -- Current Sensor/RConn1
  ib_grid/LConn1 -- Current Sensor1/RConn1
  Voltage Sensor2/RConn1 -- uc_grid/LConn1
  Current Sensor1/RConn2 -- ub/RConn1
  Voltage Sensor/LConn1 -- Current Sensor/LConn1 -- Ua/RConn1
  Current Sensor2/LConn1 -- Voltage Sensor2/LConn1 -- Uc/RConn1
  Voltage Sensor1/RConn1 -- ub_grid/LConn1
  Current Sensor/RConn2 -- ua/RConn1
  Voltage Sensor/RConn1 -- ua_grid/LConn1
  Voltage Sensor1/RConn2 -- Voltage Sensor2/RConn2 -- Voltage Sensor/RConn2 -- Electrical Reference1/LConn1
  Voltage Sensor1/LConn1 -- Current Sensor1/LConn1 -- Ub/RConn1

== system ps_25V_12kA_r/afe_abc_mod1/afe/sv_pwm ==
  duties_uvw : Inport
  Bus Selector2 : BusSelector  OutputSignals=du(k),dv(k),dw(k)
  Constant1 : Constant  Value=param.afe.behav.pwm_phase_shift_mod1
  modulator1 : Subsystem
  td2tc_1 : TransferFcn  Denominator=[param.glb_time.tc 1]
  td2tc_2 : TransferFcn  Denominator=[param.glb_time.tc 1]
  td2tc_3 : TransferFcn  Denominator=[param.glb_time.tc 1]
  gate_cmds : Outport
  wires:
  modulator1/1(gate_cmds) -> gate_cmds/1
  Constant1/1 -> modulator1/4(phase)
  Bus Selector2/1 -> td2tc_1/1  "<du(k)>"
  Bus Selector2/2 -> td2tc_2/1  "<dv(k)>"
  Bus Selector2/3 -> td2tc_3/1  "<dw(k)>"
  duties_uvw/1 -> Bus Selector2/1
  td2tc_1/1 -> modulator1/1(u)  "du(t)"
  td2tc_3/1 -> modulator1/3(w)  "dw(t)"
  td2tc_2/1 -> modulator1/2(v)  "dv(t)"

== system ps_25V_12kA_r/afe_abc_mod1/afe/three_phase_inverter_ideal_switch_based_model ==
  gate_commands : Inport
  three_phase_inverter_ideal_switch_based_model : three_phase_inverter_ideal_switch_based_model/three phase inverter ideal switch based model  Ron_ideal_switch=param.afe.ideal_switch.Rds_on  Vth=param.afe.ideal_switch.Vth  Vgamma=param.afe.ideal_switch.Vdon_diode  Rdon_diode=param.afe.ideal_switch.Rdon_diode  Csnubber=param.afe.ideal_switch.Csnubber  Rsnubber=param.afe.ideal_switch.Rsnubber
  udc(+) : PMIOPort  Side=Left
  u : PMIOPort  Port=2  Side=Right
  v : PMIOPort  Port=3  Side=Right
  udc(-) : PMIOPort  Port=4  Side=Left
  w : PMIOPort  Port=5  Side=Right
  tag scope: afe_ideal_switch_data=global
  wires:
  gate_commands/1 -> three_phase_inverter_ideal_switch_based_model/1
  three_phase_inverter_ideal_switch_based_model/1 -> [afe_ideal_switch_data]
  connections:
  three_phase_inverter_ideal_switch_based_model/RConn2 -- v/RConn1
  three_phase_inverter_ideal_switch_based_model/LConn1 -- udc(+)/RConn1
  three_phase_inverter_ideal_switch_based_model/LConn2 -- udc(-)/RConn1
  three_phase_inverter_ideal_switch_based_model/RConn1 -- u/RConn1
  three_phase_inverter_ideal_switch_based_model/RConn3 -- w/RConn1

== system ps_25V_12kA_r/afe_abc_mod1/afe/three_phase_inverter_igbt_based_with_thermal_model ==
  gate_commands : Inport
  three_phase_inverter_igbt_adv_thermal_model : three_phase_inverter_igbt_advanced_thermal_model/three_phase_inverter_igbt_adv_thermal_model  mass_heatsink_m=param.thermal.heatsink.no_weight  specific_heat_m=param.thermal.heatsink.cp  rth_switch_HA_m=param.thermal.heatsink.Rth_switch_HA  rth_switch_JH_m=param.afe.igbt.Rth_switch_JH  rth_diode_HA_m=param.afe.igbt.Rth_diode_CH  rth_diode_JH_m=param.afe.igbt.Rth_diode_JH  Rce_on_m=param.afe.igbt.Rce_on  Vce_sat_m=param.afe.igbt.Vce_sat  Vth_m=param.afe.igbt.Vth  Eon_m=param.afe.igbt.Eon  Eoff_m=param.afe.igbt.Eoff  Erec_m=param.afe.igbt.Erec  Irr_m=param.afe.igbt.Irr  Voff_sw_loss_m=param.afe.igbt.Voff_sw_losses  Ion_sw_loss_m=param.afe.igbt.Ion_sw_losses  Vdon_diode_m=param.afe.igbt.Vdon_diode  Rdon_diode_m=param.afe.igbt.Rdon_diode  Csnubber_m=param.afe.igbt.Csnubber  Rsnubber_m=param.afe.igbt.Rsnubber  JunctionTermalMass_m=param.afe.igbt.JunctionTermalMass  Tambient_m=param.thermal.heatsink.Tambient  DThs_init_m=param.thermal.heatsink.DThs_init  Lstray_module_m=param.afe.igbt.Lstray_module  Cies_m=param.afe.igbt.Cies  tc_m=param.glb_time.tc
  u : PMIOPort  Side=Right
  udc(+) : PMIOPort  Port=2  Side=Left
  v : PMIOPort  Port=3  Side=Right
  udc(-) : PMIOPort  Port=4  Side=Left
  w : PMIOPort  Port=5  Side=Right
  tag scope: afe_igbt_data=global
  wires:
  gate_commands/1 -> three_phase_inverter_igbt_adv_thermal_model/1
  three_phase_inverter_igbt_adv_thermal_model/1 -> [afe_igbt_data]
  connections:
  three_phase_inverter_igbt_adv_thermal_model/RConn1 -- u/RConn1
  three_phase_inverter_igbt_adv_thermal_model/LConn2 -- udc(-)/RConn1
  three_phase_inverter_igbt_adv_thermal_model/LConn1 -- udc(+)/RConn1
  three_phase_inverter_igbt_adv_thermal_model/RConn2 -- v/RConn1
  three_phase_inverter_igbt_adv_thermal_model/RConn3 -- w/RConn1

== system ps_25V_12kA_r/afe_abc_mod1/afe/three_phase_inverter_mosfet_based_with_thermal_model ==
  gate_commands : Inport
  three phase inverter mosfet based with thermal model : three_phase_inverter_mosfet_based_with_thermal_model/three phase inverter mosfet based with thermal model  mass_heatsink_m=0.2  specific_heat_m=880  rth_mosfet_HA_m=0.02  rth_mosfet_JH_m=0.075  Rds_on_m=0.00185  Vth_m=7.5  Eon_m=0.077  Eoff_m=0.108  Voff_sw_loss_m=1300  Ion_sw_loss_m=1000  Vdon_diode_m=4  Rdon_diode_m=0.00185  JunctionTermalMass_m=2  Tambient_m=40  DThs_init_m=0
  u : PMIOPort  Side=Right
  udc(+) : PMIOPort  Port=2  Side=Left
  v : PMIOPort  Port=3  Side=Right
  udc(-) : PMIOPort  Port=4  Side=Left
  w : PMIOPort  Port=5  Side=Right
  wires:
  gate_commands/1 -> three phase inverter mosfet based with thermal model/1
  connections:
  three phase inverter mosfet based with thermal model/RConn3 -- w/RConn1
  three phase inverter mosfet based with thermal model/RConn2 -- v/RConn1
  three phase inverter mosfet based with thermal model/LConn1 -- udc(+)/RConn1
  three phase inverter mosfet based with thermal model/LConn2 -- udc(-)/RConn1
  three phase inverter mosfet based with thermal model/RConn1 -- u/RConn1

== system ps_25V_12kA_r/afe_abc_mod1/brake/Rbrake ==
  PS-Simulink Converter2 : nesl_utility/PS-Simulink Converter  PhysicalDomain=network_engine_domain  SubClassName=ps_output  LeftPortType=input  RightPortType=output  PseudoPeriodic=off  Frequencies=[]  VectorFormat=1-D array  Unit=degC  AffineConversion=off
  PS-Simulink Converter3 : nesl_utility/PS-Simulink Converter  PhysicalDomain=network_engine_domain  SubClassName=ps_output  LeftPortType=input  RightPortType=output  PseudoPeriodic=off  Frequencies=[]  VectorFormat=1-D array  Unit=W  AffineConversion=off
  Rbrake_thermal : Scope  NumInputPorts=2
      settings: ActiveDisplayYMinimum=-0.005623823950706707  ActiveDisplayYMaximum=0.05061441555636037  DataLoggingVariableName=ScopeData33
  Resistor1 : ee_lib/Passive/Resistor  R=param.afe.hw.Rbrake Ohm  enable_R_tol=ee.enum.toleranceApplication.none  R_tol=5  tol_distribution=ee.enum.toleranceDistribution.uniform  nSigma=4  enable_operating_limits=ee.enum.enable.no  operating_limit_action=ee.enum.passive.reportOpLim.warn  power_rating=1 W  max_working_voltage=100 V  noise_mode=ee.enum.sources.noise.Disabled  Tdevice=25 degC  sample_time=1e-3 s  repeatability=ee.enum.ic.repeatability.notRepeatable  user_seed=0  auto_seed=1811450916  power_derating_T1=70 degC  power_derating_T2=155 degC  operating_temperature_range_vec=[-50, 150] degC  alpha=3.93e-3 1/K  Tmeas=25 degC  thermal_mass=100 J/K  temperature_specify=off  temperature_priority=High  temperature=298.15 K  temperature_nominal_specify=off  temperature_nominal_value=1  temperature_nominal_unit=K
  Tambient : fl_lib/Thermal/Thermal Sources/Temperature Source  temperature=param.thermal.Tambient degC
  Temperature Sensor1 : fl_lib/Thermal/Thermal Sensors/Temperature Sensor  temperature_measure=foundation.enum.MeasurementReference.difference
  To Workspace1 : ToWorkspace  VariableName=RbrakePowerFlow_mod1_sim  SampleTime=param.glb_time.tc
      settings: MaxDataPoints=param.glb_time.Nc
  To Workspace10 : ToWorkspace  VariableName=RbrakeTemperature_mod1_sim  SampleTime=param.glb_time.tc
      settings: MaxDataPoints=param.glb_time.Nc
  heatsink_C : fl_lib/Thermal/Thermal Elements/Thermal Mass  mass_type=foundation.enum.constant_variable.constant  mass=40 kg  sp_heat=505 J/(K*kg)  mass_min=1e-6 kg  num_ports=foundation.enum.numPorts2.one  m_specify=off  m_priority=High  m=1 kg  m_nominal_specify=off  m_nominal_value=1  m_nominal_unit=kg  T_specify=on  T_priority=High  T=param.thermal.DThs_init+param.thermal.Tambient degC  T_nominal_specify=off  T_nominal_value=1  T_nominal_unit=K  Q_specify=off  Q_priority=High  Q=0 W  Q_nominal_specify=off  Q_nominal_value=1  Q_nominal_unit=W
  power_losses_switch : fl_lib/Thermal/Thermal Sensors/Heat Flow Rate Sensor
  switch_heatsink : fl_lib/Thermal/Thermal Elements/Thermal Resistance  resistance=300/48e3 K/W  T_specify=off  T_priority=High  T=0 deltadegC  T_nominal_specify=off  T_nominal_value=1  T_nominal_unit=K  Q_specify=off  Q_priority=None  Q=0 W  Q_nominal_specify=off  Q_nominal_value=1  Q_nominal_unit=W
  A : PMIOPort  Side=Left
  B : PMIOPort  Port=2  Side=Right
  wires:
  PS-Simulink Converter2/1 -> To Workspace10/1, Rbrake_thermal/1  "RbrakeTemperature"
  PS-Simulink Converter3/1 -> To Workspace1/1, Rbrake_thermal/2  "RbrakePowerFlow"
  connections:
  Resistor1/LConn1 -- A/RConn1
  Resistor1/RConn1 -- B/RConn1
  Tambient/LConn1 -- Temperature Sensor1/RConn1 -- switch_heatsink/RConn1
  Temperature Sensor1/LConn1 -- power_losses_switch/RConn2 -- heatsink_C/LConn1 -- switch_heatsink/LConn1
  Temperature Sensor1/RConn2 -- PS-Simulink Converter2/LConn1
  power_losses_switch/LConn1 -- Resistor1/LConn2
  power_losses_switch/RConn1 -- PS-Simulink Converter3/LConn1

== system ps_25V_12kA_r/afe_abc_mod1/brake/switch_1 ==
  Capacitor : fl_lib/Electrical/Electrical Elements/Capacitor  c=param.afe.ideal_switch.Csnubber F  r=param.afe.ideal_switch.Rsnubber Ohm  g=0 1/Ohm  i_specify=off  i_priority=None  i=0 A  i_nominal_specify=off  i_nominal_value=1  i_nominal_unit=A  v_specify=off  v_priority=None  v=0 V  v_nominal_specify=off  v_nominal_value=1  v_nominal_unit=V  vc_specify=off  vc_priority=High  vc=0 V  vc_nominal_specify=off  vc_nominal_value=1  vc_nominal_unit=V
  Diode : fl_lib/Electrical/Electrical Elements/Diode  Vf=param.afe.ideal_switch.Vgamma V  Ron=param.afe.ideal_switch.Rdon_diode Ohm  Goff=1e-8 1/Ohm  i_specify=off  i_priority=None  i=0 A  i_nominal_specify=off  i_nominal_value=1  i_nominal_unit=A  v_specify=off  v_priority=None  v=0 V  v_nominal_specify=off  v_nominal_value=1  v_nominal_unit=V
  C : PMIOPort  Side=Left
  E : PMIOPort  Port=2  Side=Right
  connections:
  Diode/LConn1 -- Capacitor/RConn1 -- E/RConn1
  Diode/RConn1 -- C/RConn1 -- Capacitor/LConn1

== system ps_25V_12kA_r/afe_abc_mod1/brake/switch_2 ==
  Capacitor : fl_lib/Electrical/Electrical Elements/Capacitor  c=param.afe.ideal_switch.Csnubber F  r=param.afe.ideal_switch.Rsnubber Ohm  g=0 1/Ohm  i_specify=off  i_priority=None  i=0 A  i_nominal_specify=off  i_nominal_value=1  i_nominal_unit=A  v_specify=off  v_priority=None  v=0 V  v_nominal_specify=off  v_nominal_value=1  v_nominal_unit=V  vc_specify=off  vc_priority=High  vc=0 V  vc_nominal_specify=off  vc_nominal_value=1  vc_nominal_unit=V
  Diode : fl_lib/Electrical/Electrical Elements/Diode  Vf=param.afe.ideal_switch.Vgamma V  Ron=param.afe.ideal_switch.Rdon_diode Ohm  Goff=1e-8 1/Ohm  i_specify=off  i_priority=None  i=0 A  i_nominal_specify=off  i_nominal_value=1  i_nominal_unit=A  v_specify=off  v_priority=None  v=0 V  v_nominal_specify=off  v_nominal_value=1  v_nominal_unit=V
  Switch : fl_lib/Electrical/Electrical Elements/Switch  R_closed=param.afe.ideal_switch.Rds_on Ohm  G_open=1e-8 1/Ohm  Threshold=7.5  i_specify=off  i_priority=None  i=0 A  i_nominal_specify=off  i_nominal_value=1  i_nominal_unit=A  v_specify=off  v_priority=None  v=0 V  v_nominal_specify=off  v_nominal_value=1  v_nominal_unit=V
  G : PMIOPort  Side=Left
  C : PMIOPort  Port=2  Side=Left
  E : PMIOPort  Port=3  Side=Right
  connections:
  Switch/RConn2 -- C/RConn1 -- Capacitor/LConn1 -- Diode/RConn1
  Switch/RConn1 -- G/RConn1
  Switch/LConn1 -- E/RConn1 -- Capacitor/RConn1 -- Diode/LConn1

== system ps_25V_12kA_r/full_bridge_converter/full_bridge_converter_with_iso/full_bridge ==
  gate_commands : Inport
  full-bridge_ideal_switch_based : Subsystem
  full-bridge_mosfet_based_ with_thermal_model_zvs : Subsystem  Commented=on
  full_bridge_igbt_adv_thermal_model : Subsystem  Commented=on
  uac_1(+) : PMIOPort  Side=Left
  uac_1(-) : PMIOPort  Port=2  Side=Left
  Udc(+) : PMIOPort  Port=3  Side=Right
  Udc(-) : PMIOPort  Port=4  Side=Right
  wires:
  gate_commands/1 -> full-bridge_mosfet_based_ with_thermal_model_zvs/1(gate_commands), full_bridge_igbt_adv_thermal_model/1(gate_commands), full-bridge_ideal_switch_based/1(gate_commands)
  connections:
  full_bridge_igbt_adv_thermal_model/RConn2 -- full-bridge_mosfet_based_ with_thermal_model_zvs/RConn2 -- uac_1(-)/RConn1 -- full-bridge_ideal_switch_based/RConn2
  Udc(-)/RConn1 -- full-bridge_mosfet_based_ with_thermal_model_zvs/LConn2 -- full_bridge_igbt_adv_thermal_model/LConn2 -- full-bridge_ideal_switch_based/LConn2
  Udc(+)/RConn1 -- full-bridge_mosfet_based_ with_thermal_model_zvs/LConn1 -- full_bridge_igbt_adv_thermal_model/LConn1 -- full-bridge_ideal_switch_based/LConn1
  full_bridge_igbt_adv_thermal_model/RConn1 -- full-bridge_mosfet_based_ with_thermal_model_zvs/RConn1 -- uac_1(+)/RConn1 -- full-bridge_ideal_switch_based/RConn1

== system ps_25V_12kA_r/full_bridge_converter/full_bridge_converter_with_iso/scopes ==
  psfbc TR i2/i1 : Scope  NumInputPorts=2
      settings: SampleTime=param.glb_time.tc  ActiveDisplayYMinimum=-1133.8385972087863  ActiveDisplayYMaximum=1130.02633442417  DataLoggingVariableName=ScopeData13
  psfbc TR u2/u1 : Scope  NumInputPorts=2
      settings: SampleTime=param.glb_time.tc  ActiveDisplayYMinimum=-1550.0820677220172  ActiveDisplayYMaximum=1550.0802549877285  DataLoggingVariableName=ScopeData4
  psfbc current output/input : Scope  NumInputPorts=2
      settings: SampleTime=param.glb_time.tc  ActiveDisplayYMinimum=11712.561102123631  ActiveDisplayYMaximum=12410.217552147782  DataLoggingVariableName=ScopeData8
  psfbc outputs modA : Scope  NumInputPorts=2
      settings: SampleTime=param.glb_time.tc  ActiveDisplayYMinimum=-1385.5793837278463  ActiveDisplayYMaximum=12470.126167619435  DataLoggingVariableName=ScopeData6
  psfbc voltage input/output : Scope  NumInputPorts=2
      settings: SampleTime=param.glb_time.tc  ActiveDisplayYMinimum=-130.82892689030524  ActiveDisplayYMaximum=1177.4603420127473  DataLoggingVariableName=ScopeData10
  psfbc_analysis : Scope  NumInputPorts=4
      settings: SampleTime=param.glb_time.tc  ActiveDisplayYMinimum=-3614.5429375394424  ActiveDisplayYMaximum=8289.5390361005484  DataLoggingVariableName=ScopeData5
  wires:
  [psfbc_voltage_input] -> psfbc voltage input/output/1  "psfbc_voltage_input_modA"
  [psfbc_current_output] -> psfbc current output/input/1  "psfbc_current_output_modA"
  [psfbc_voltage_output] -> psfbc voltage input/output/2  "psfbc_voltage_output_modA"
  [psfbc_current_input] -> psfbc current output/input/2  "psfbc_current_input_modA"
  [i2_psfbc_transformer_modA] -> psfbc TR i2/i1/1  "i2_psfbc_transformer_modA"
  [i1_psfbc_transformer] -> psfbc TR i2/i1/2  "i1_psfbc_transformer_modA"
  [u2_psfbc_transformer_modA] -> psfbc TR u2/u1/1  "u2_psfbc_transformer_modA"
  [u1_psfbc_transformer] -> psfbc TR u2/u1/2  "u1_psfbc_transformer_modA"
  [psfbc_voltage_output] -> psfbc outputs modA/2  "psfbc_voltage_output"
  [psfbc_current_output] -> psfbc outputs modA/1  "psfbc_current_output"
  [i2_psfbc_transformer_modA] -> psfbc_analysis/1  "i2_psfbc_transformer_modA"
  [i1_psfbc_transformer] -> psfbc_analysis/2  "i1_psfbc_transformer_modA"
  [u2_psfbc_transformer_modA] -> psfbc_analysis/3  "u2_psfbc_transformer_modA"
  [u1_psfbc_transformer] -> psfbc_analysis/4  "u1_psfbc_transformer_modA"

== system ps_25V_12kA_r/full_bridge_converter/full_bridge_converter_with_iso/trafo_rectifier ==
  rectifiers : Subsystem
  transformers : Subsystem
  uac_1(+) : PMIOPort  Side=Left
  udc_load(+) : PMIOPort  Port=2  Side=Right
  uac_1(-) : PMIOPort  Port=3  Side=Left
  udc_load(-) : PMIOPort  Port=4  Side=Right
  connections:
  rectifiers/RConn1 -- udc_load(+)/RConn1
  rectifiers/RConn2 -- udc_load(-)/RConn1
  uac_1(-)/RConn1 -- transformers/LConn2
  uac_1(+)/RConn1 -- transformers/LConn1
  transformers/RConn1 -- rectifiers/LConn1
  transformers/RConn2 -- rectifiers/LConn2
  transformers/RConn3 -- rectifiers/LConn3
  transformers/RConn4 -- rectifiers/LConn4
  transformers/RConn5 -- rectifiers/LConn5

== system ps_25V_12kA_r/full_bridge_converter/phase_shift_full_bridge_ctrl/references ==
  Rate Limiter : RateLimiter  RisingSlewLimit=param.psfbc.hw.idc2_nom*10  FallingSlewLimit=-param.psfbc.hw.idc2_nom*10  SampleTimeMode=inherited
  Vout_dc_nom : Step  Time=0.025  FinalValue=param.psfbc.hw.idc2_nom  SampleTime=0
  vout_ref : Outport
  wires:
  Rate Limiter/1 -> vout_ref/1
  Vout_dc_nom/1 -> Rate Limiter/1

== system ps_25V_12kA_r/full_bridge_converter/phase_shift_full_bridge_ctrl/sampling_i_filter1 ==
  in : Inport
  1/Ti3 : Gain  Gain=1/param.psfbc.hw.idc2_bez  OutDataTypeStr=double  SaturateOnIntegerOverflow=on  ParamDataTypeStr=Inherit: Same as input
  out_pu : Outport
  wires:
  in/1 -> 1/Ti3/1
  1/Ti3/1 -> out_pu/1

== system ps_25V_12kA_r/full_bridge_converter/phase_shift_full_bridge_ctrl/sampling_i_filter2 ==
  in : Inport
  1/Ti3 : Gain  Gain=1/param.psfbc.hw.idc1_bez  OutDataTypeStr=double  SaturateOnIntegerOverflow=on  ParamDataTypeStr=Inherit: Same as input
  out_pu : Outport
  wires:
  1/Ti3/1 -> out_pu/1
  in/1 -> 1/Ti3/1

== system ps_25V_12kA_r/full_bridge_converter/phase_shift_full_bridge_ctrl/sampling_v_filter1 ==
  in : Inport
  1/Ti3 : Gain  Gain=1/param.psfbc.hw.udc2_bez  OutDataTypeStr=double  SaturateOnIntegerOverflow=on  ParamDataTypeStr=Inherit: Same as input
  out_pu : Outport
  wires:
  in/1 -> 1/Ti3/1
  1/Ti3/1 -> out_pu/1

== system ps_25V_12kA_r/full_bridge_converter/phase_shift_full_bridge_ctrl/sampling_v_filter2 ==
  in : Inport
  1/Ti3 : Gain  Gain=1/param.psfbc.hw.idc2_nom  OutDataTypeStr=double  SaturateOnIntegerOverflow=on  ParamDataTypeStr=Inherit: Same as input
  Saturation : Saturate  UpperLimit=1  LowerLimit=0  OutDataTypeStr=double
  out_pu : Outport
  wires:
  in/1 -> 1/Ti3/1
  1/Ti3/1 -> Saturation/1
  Saturation/1 -> out_pu/1
